simulink model "testrig_AirOilPiston"  (R2026b)
settings: Solver=daessc  StopTime=25  MaxStep=1e-3  AbsTol=1e-3
PreLoadFcn:
  | Spring = VDatabase.Spring.SUV_Landy_TA2PR_AirOilPiston_A1;
  | mass_sprung = 436.5;
  | load testrig_AirOilPiston_roughroad
PostLoadFcn:
  | warning off Simulink:blocks:TDelayBufferTooSmall
undefined symbols (not defined in the file or in its folder): Triangle
libraries: fl_lib x10, nesl_utility x5, simulink x4, Spring_AirOilPiston x1, testrig_AirOilPiston_lib x1
settings Model: Creator=Glenn  LastModifiedBy=smiller
settings SolverCC: AutoScaleAbsTol=off  MaxConsecutiveMinStep=5
settings DataIOCC: ReturnWorkspaceOutputs=off  SignalLoggingName=logsout_testrig_AirOilPiston
settings SimscapeCC: SimscapeLogLimitData=off  SimscapeLogName=simlog_testrig_AirOilPiston  SimscapeLogType=all  SimscapeUseEnergyAccounting=off

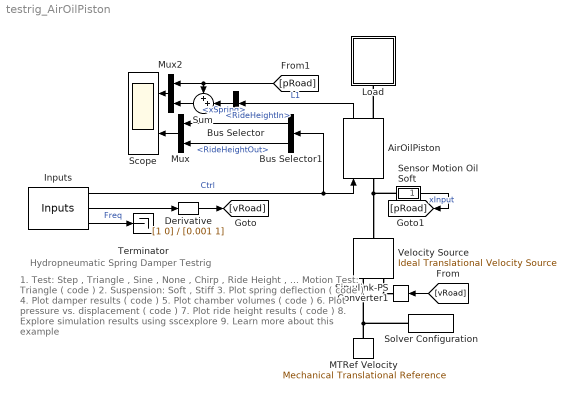
== system testrig_AirOilPiston ==
  note: 1. Test: Step , Triangle , Sine , None , Chirp , Ride Height , ... Motion Test: Triangle ( code )
      | 2. Suspension: Soft , Stiff
      | 3. Plot spring deflection ( code )
      | 4. Plot damper results ( code )
      | 5. Plot chamber volumes ( code )
      | 6. Plot pressure vs. displacement ( code )
      | 7. Plot ride height results ( code )
      | 8. Explore simulation results using sscexplore
      | 9. Learn more about this example
  note: Hydropneumatic Spring Damper Testrig
  AirOilPiston : Spring_AirOilPiston/AirOilPiston  spr_hp_top=Spring.sTop.Value*0  spr_hp_bot=Spring.sBottom.Value*0  t_ambient=Spring.Spring.TAmbient.Value  gspr_gas_properties=Spring.Spring.GasProperties  strut_oil_properties=Spring.Strut.OilProperties  gas_chamber_soft_area=Spring.Spring.GasSoft.A.Value  gas_chamber_stiff_area=Spring.Spring.GasStiff.A.Value  gas_chamber_soft_deadvol=Spring.Spring.GasSoft.volDead.Value  gas_chamber_stiff_deadvol=Spring.Spring.GasStiff.volDead.Value  gspr_mass_soft=Spring.Spring.GasSoft.mPiston.Value  gspr_mass_stiff=Spring.Spring.GasStiff.mPiston.Value  gspr_damping_soft=Spring.Spring.GasSoft.b.Value  gspr_damping_stiff=Spring.Spring.GasStiff.b.Value  gas_chamber_soft_x0=Spring.Spring.GasSoft.xInit.Value  gas_chamber_stiff_x0=Spring.Spring.GasStiff.xInit.Value  gas_chamber_soft_p0=Spring.Spring.GasSoft.pInit.Value  gas_chamber_stiff_p0=Spring.Spring.GasStiff.pInit.Value  gspr_cwall_soft=Spring.Spring.GasSoft.CWall.Value  gspr_cwall_stiff=Spring.Spring.GasStiff.CWall.Value  oil_chamber_soft_area=Spring.Spring.OilSoft.A.Value  oil_chamber_stiff_area=Spring.Spring.OilStiff.A.Value  oil_chamber_soft_deadvol=Spring.Spring.OilSoft.volDead.Value  oil_chamber_stiff_deadvol=Spring.Spring.OilStiff.volDead.Value  oil_chamber_soft_x0=Spring.Spring.OilSoft.xInit.Value  oil_chamber_stiff_x0=Spring.Spring.OilStiff.xInit.Value  oil_chamber_soft_p0=Spring.Spring.OilSoft.pInit.Value  oil_chamber_stiff_p0=Spring.Spring.OilStiff.pInit.Value  gsprv_smax_soft=Spring.Spring.ValveSoft.xMaxOpen.Value  gsprv_smax_stiff=Spring.Spring.ValveStiff.xMaxOpen.Value  gsprv_delsmax_soft=Spring.Spring.ValveSoft.xCloseToOpen.Value  gsprv_delsmax_stiff=Spring.Spring.ValveStiff.xCloseToOpen.Value  gsprv_arealeak_soft=Spring.Spring.ValveSoft.areaLeak.Value  gsprv_arealeak_stiff=Spring.Spring.ValveStiff.areaLeak.Value  gsprv_areamax_soft=Spring.Spring.ValveSoft.aMax.Value  gsprv_areamax_stiff=Spring.Spring.ValveStiff.aMax.Value  gsprv_cd_soft=Spring.Spring.ValveSoft.Cd.Value  gsprv_cd_stiff=Spring.Spring.ValveStiff.Cd.Value  gsprv_smooth_soft=Spring.Spring.ValveSoft.smoothFactor.Value  gsprv_smooth_stiff=Spring.Spring.ValveStiff.smoothFactor.Value  gsprva_stroke_soft=Spring.Spring.ValveActuatorSoft.xStroke.Value  gsprva_stroke_stiff=Spring.Spring.ValveActuatorStiff.xStroke.Value  gsprva_ton_soft=Spring.Spring.ValveActuatorSoft.tOn.Value  gsprva_ton_stiff=Spring.Spring.ValveActuatorStiff.tOn.Value  gsprva_toff_soft=Spring.Spring.ValveActuatorSoft.tOff.Value  gsprva_toff_stiff=Spring.Spring.ValveActuatorStiff.tOff.Value  strut_deadvol=Spring.Strut.volDead.Value  strut_area=Spring.Strut.A.Value  strut_x0=Spring.Strut.xInit.Value  strut_frc_colfrc=Spring.Strut.Friction.fCoulomb.Value  strut_frc_brkfrc=Spring.Strut.Friction.fBreakaway.Value  strut_frc_brkvel=Spring.Strut.Friction.vBreakaway.Value  strut_frc_visccoeff=Spring.Strut.Friction.mu.Value  strut_p0=Spring.Strut.pInit.Value  bs_lim_upper=Spring.Endstop.xMax.Value  bs_lim_lower=Spring.Endstop.xMin.Value  bs_k_upper=Spring.Endstop.KxMax.Value  bs_k_lower=Spring.Endstop.KxMin.Value  bs_b_upper=Spring.Endstop.dxMax.Value  bs_b_lower=Spring.Endstop.dxMin.Value  bs_region=Spring.Endstop.xTransition.Value  p_diff_TLU_constant=Spring.Damper.Orifice.pDiff.Value  vol_flow_TLU_constant=Spring.Damper.Orifice.q.Value  dpr_restrarea_comp=Spring.Damper.RestrictionComp.A.Value  dpr_restrarea_reb=Spring.Damper.RestrictionReb.A.Value  dpr_cd_comp=Spring.Damper.RestrictionComp.Cd.Value  dpr_cd_reb=Spring.Damper.RestrictionReb.Cd.Value  dpr_prv_psetdiff_comp=Spring.Damper.PRVComp.pDiff.Value  dpr_prv_psetdiff_reb=Spring.Damper.PRVReb.pDiff.Value  dpr_prv_prange_comp=Spring.Damper.PRVComp.pRange.Value  dpr_prv_prange_reb=Spring.Damper.PRVReb.pRange.Value  dpr_prv_areamax_comp=Spring.Damper.PRVComp.A.Value  dpr_prv_areamax_reb=Spring.Damper.PRVReb.A.Value  dpr_prv_cd_comp=Spring.Damper.PRVComp.Cd.Value  dpr_prv_cd_reb=Spring.Damper.PRVReb.Cd.Value  dpr_cvdvalve_cmpos=Spring.CVDValve.Orifice.x.Value  dpr_cvdvalve_orifice_area=Spring.CVDValve.Orifice.A.Value  dpr_cvdvalve_orifice_pdiff=Spring.CVDValve.Orifice.pDiff.Value  dpr_cvdvalve_pcv_areamax=Spring.CVDValve.PCValve.AMax.Value  dpr_cvdvalve_pcv_prange=Spring.CVDValve.PCValve.pRange.Value  dpr_cvdvalve_arealeak=Spring.CVDValve.PCValve.ALeak.Value  dpr_cvdvalve_cd=Spring.CVDValve.PCValve.Cd.Value  dpr_cvdvalve_act_ts=Spring.CVDValve.tFilt.Value  rh_srcpressure=Spring.RideHeight.pSource.Value  rh_fcv_cmpos_inlet=Spring.RideHeight.OrificeInlet.x.Value  rh_fcv_cmpos_outlet=Spring.RideHeight.OrificeOutlet.x.Value  rh_fcv_orificearea_inlet=Spring.RideHeight.OrificeInlet.A.Value  rh_fcv_orificearea_outlet=Spring.RideHeight.OrificeOutlet.A.Value  rh_fcv_orificepdiff_inlet=Spring.RideHeight.OrificeInlet.pDiff.Value  rh_fcv_orificepdiff_outlet=Spring.RideHeight.OrificeOutlet.pDiff.Value  rh_fcv_pcprange_inlet=Spring.RideHeight.PCValveInlet.pRange.Value  rh_fcv_pcprange_outlet=Spring.RideHeight.PCValveOutlet.pRange.Value  rh_fcv_pcamax_inlet=Spring.RideHeight.PCValveInlet.AMax.Value  rh_fcv_pcamax_outlet=Spring.RideHeight.PCValveOutlet.AMax.Value  rh_fcv_arealeak_inlet=Spring.RideHeight.PCValveInlet.ALeak.Value  rh_fcv_arealeak_outlet=Spring.RideHeight.PCValveOutlet.ALeak.Value  rh_fcv_cd_inlet=Spring.RideHeight.PCValveInlet.Cd.Value  rh_fcv_cd_outlet=Spring.RideHeight.PCValveOutlet.Cd.Value  rh_fcv_smooth_inlet=Spring.RideHeight.PCValveInlet.smoothFactor.Value  rh_fcv_smooth_outlet=Spring.RideHeight.PCValveOutlet.smoothFactor.Value  rh_fcv_tfilt_inlet=Spring.RideHeight.PCValveInlet.tFilt.Value  rh_fcv_tfilt_outlet=Spring.RideHeight.PCValveOutlet.tFilt.Value
  Bus Selector : BusSelector  OutputSignals=xSpring
  Bus Selector1 : BusSelector  OutputSignals=RideHeightIn,RideHeightOut
  Derivative : TransferFcn  Numerator=[1 0]  Denominator=[0.001 1]
  Inputs : testrig_AirOilPiston_lib/Inputs  popup_suspension_stiffness=Soft  popup_rh_test_seq=None  cvd_value=1  popup_roadpz_test_type=Step  pAmp=0.05  tPer=4  nCyc=50  nCycSet=1  chirpFreqFinish=10  chirpFreqStart=0.5  chirpTimeFinish=25  chirpTimeStart=5  spdkmh=10  roughTimeStart=5
      settings: AttributesFormatString=|
      | Road Height: %<popup_roadpz_test_type>
      | Suspension: %<popup_suspension_stiffness>
      | Ride Height: %<popup_rh_test_seq>
  Load : Subsystem  Variant=on  VariantControlMode=label  VariantControl=Mass  LabelModeActiveChoice=Mass  mask{popup_load_type=Mass}
      mask prompts: popup_load_type "Load Type"
      mask init:
      | bh = gcb;
      | set_param(gcb,'LabelModeActiveChoice',get_param(bh,'popup_load_type'));
      settings: AttributesFormatString=%<popup_load_type>
      mask TypeOptions popup_load_type: Mass | Motion
      mask Display: disp(' ')
  MTRef Velocity : fl_lib/Mechanical/Translational Elements/Mechanical Translational Reference
  Mux : Mux  Inputs=2
  Mux2 : Mux  Inputs=2
  Scope : Scope  NumInputPorts=2
      settings: ActiveDisplayYMinimum=-0.07527  ActiveDisplayYMaximum=0.08974
  Sensor Motion Oil Soft : Subsystem
  Simulink-PS Converter1 : nesl_utility/Simulink-PS Converter  PhysicalDomain=network_engine_domain  SubClassName=ps_input  LeftPortType=input  RightPortType=output  PseudoPeriodic=off  Frequencies=[]  NoiseDistribution=none  NoiseParameters=[]  Unit=m/s  AffineConversion=off  FilteringAndDerivatives=provide  SimscapeFilterOrder=1  InputFilterTimeConstant=0.001  UdotUserProvided=0
  Solver Configuration : nesl_utility/Solver Configuration  PhysicalDomain=network_engine_domain  SubClassName=solver  LeftPortType=input  RightPortType=generic  Tones=[]  Harmonics=[]  SimulateNoise=off  Profile=off  UseLocalSampling=off  EnableSwitchedLinearOptims=on  FrequencyDomain=off  UseCCode=off  RelTol=0.001  AbsTol=0.001  MinStep=1e-09  ToWorkspace=off  RevertToSquareIcSolve=off  NumHomotopyIterations=100  PhasorMode=off  PhasorModeNumHarmonics=1  ConsistencySolver=NEWTON_FTOL  CanonicalOrdering=UNORDERED  OptimizeIntermediates=UNOPTIMIZED  MulticoreSolverChoice=BACKWARD_EULER  IndexReductionMethod=DerivativeReplacement  DoDC=off  ResidualTolerance=1e-09  ConsistencyTolSource=GLOBAL  ConsistencyAbsTol=0.001  ConsistencyRelTol=0.001  ConsistencyTolFactor=0.001  UseLocalSolver=off  LocalSolverChoice=NE_BACKWARD_EULER_ADVANCER  ResolveIndetEquations=on  FunctionEvalNumThread=1  LocalSolverSampleTime=0.001  DoFixedCost=off  MaxNonlinIter=3  MaxModeIter=2  ComputeImpulses=off  ImpulseIterations=2  LinearAlgebra=auto  LinearAlgebraNumThread=0  EquationFormulation=NE_TIME_EF  DelaysMemoryBudget=1024  AutomaticFiltering=on  FilteringTimeConstant=0.001  PartitionStorageMethod=AS_NEEDED  PartitionMemoryBudget=1024  PartitionMethod=BALANCED  MultibodyUseLocalSolver=off  MultibodyLocalSolverChoice=ODE1  MultibodyLocalSolverSampleTime=0.001
  Sum : Sum  Inputs=++|
  Terminator : Terminator
  Velocity Source : fl_lib/Mechanical/Mechanical Sources/Ideal Translational Velocity Source
  wires:
  AirOilPiston/1 -> Bus Selector/1  "L1"
  Bus Selector/1 -> Sum/2  "<xSpring>"
  Mux/1 -> Scope/2
  Bus Selector1/1 -> Mux/1  "<RideHeightIn>"
  Bus Selector1/2 -> Mux/2  "<RideHeightOut>"
  Inputs/2 -> Derivative/1
  [vRoad] -> Simulink-PS Converter1/1
  Inputs/1 -> Bus Selector1/1, AirOilPiston/1  "Ctrl"
  Mux2/1 -> Scope/1
  Sensor Motion Oil Soft/1(P) -> [pRoad]  "xInput"
  Derivative/1 -> [vRoad]
  [pRoad] -> Sum/1, Mux2/1
  Sum/1 -> Mux2/2
  Inputs/3 -> Terminator/1  "Freq"
  connections:
  Sensor Motion Oil Soft/LConn1 -- AirOilPiston/LConn1 -- Velocity Source/LConn1
  MTRef Velocity/LConn1 -- Solver Configuration/RConn1 -- Velocity Source/RConn2
  Velocity Source/RConn1 -- Simulink-PS Converter1/RConn1
  AirOilPiston/RConn1 -- Load/LConn1

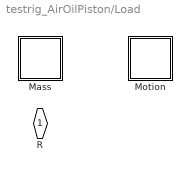
== system testrig_AirOilPiston/Load ==
  Mass : Subsystem  VariantControl=Mass
  Motion : Subsystem  VariantControl=Motion  mask{popup_signalType=Triangle, pAmp=0.05, tPer=3, nCyc=50, nCycSet=1, chirpFreqFinish=10, chirpFreqStart=0.5, chirpTimeFinish=20, chirpTimeStart=5}
      mask prompts: popup_signalType "Signal Type"; pAmp "Amplitude"; tPer "Period"; nCyc "Number of Cycles per Set"; nCycSet "Number of Cycles to Settle"; chirpFreqFinish "Chirp Freq Finish (Hz)"; chirpFreqStart "Chirp Freq Start (Hz)"; chirpTimeFinish "Chirp Time Finish (sec)"; chirpTimeStart "Chirp Start Delay (sec)"
      mask TypeOptions popup_signalType: Spring Extension Velocity/popup_signalType
      mask Callback popup_signalType:
      | bh = gcb;
      | maskObj = Simulink.Mask.get(bh); % Get the mask object of the current block
      | 
      | % Handles for parameter visibility
      | chFrSt_h  = maskObj.getParameter('chirpFreqStart'); % Get the parameter to hide
      | chFrFi_h  = maskObj.getParameter('chirpFreqFinish'); % Get the parameter to hide
      | chTiSt_h  = maskObj.getParameter('chirpTimeStart'); % Get the parameter to hide
      | chTiFi_h  = maskObj.getParameter('chirpTimeFinish'); % Get the parameter to hide
      | 
      | tPer_h    = maskObj.getParameter('tPer');    % Get the parameter to hide
      | nCycSet_h = maskObj.getParameter('nCycSet'); % Get the parameter to hide
      | nCyc_h    = maskObj.getParameter('nCyc'); % Get the parameter to hide
      | 
      | % Check the value of ControlParam
      | controlParamValue = get_param(bh, 'popup_signalType');
      | 
      | chFrSt_h.Visible   = 'off';
      | chFrFi_h.Visible   = 'off';
      | chTiFi_h.Visible   = 'off';
      | chTiSt_h.Visible   = 'off';
      | tPer_h.Visible     = 'on';
      | nCycSet_h.Visible  = 'on';
      | nCyc_h.Visible     = 'on';
      | 
      | if(strcmp(controlParamValue, 'Chirp'))
      |     chFrSt_h.Visible  = 'on';
      |     chFrFi_h.Visible  = 'on';
      |     chTiSt_h.Visible  = 'on';
      |     chTiFi_h.Visible  = 'on';
      | 
      |     tPer_h.Visible    = 'off';
      |     nCycSet_h.Visible = 'off';
      |     nCyc_h.Visible    = 'off';
      | end
      mask TypeOptions pAmp: Spring Extension Velocity/vAmp
      mask TypeOptions tPer: Spring Extension Velocity/tPer
      mask TypeOptions nCyc: Spring Extension Velocity/nCyc
      mask TypeOptions nCycSet: Spring Extension Velocity/nCycSet
      mask TypeOptions chirpFreqFinish: Spring Extension Velocity/chirpFreqFinish
      mask TypeOptions chirpFreqStart: Spring Extension Velocity/chirpFreqStart
      mask TypeOptions chirpTimeFinish: Spring Extension Velocity/chirpTimeFinish
      mask TypeOptions chirpTimeStart: Spring Extension Velocity/chirpTimeStart
  R : PMIOPort  Side=Left

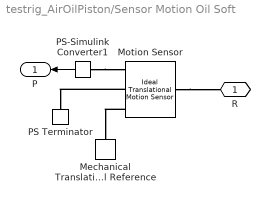
== system testrig_AirOilPiston/Sensor Motion Oil Soft ==
  Mechanical Translational Reference : fl_lib/Mechanical/Translational Elements/Mechanical Translational Reference
  Motion Sensor : fl_lib/Mechanical/Mechanical Sensors/Ideal Translational Motion Sensor  reference=foundation.enum.MeasurementReference.difference  acceleration_port=false  velocity_port=true  position_port=true  offset=0 m
  PS Terminator : fl_lib/Physical Signals/Sinks/PS Terminator
  PS-Simulink Converter1 : nesl_utility/PS-Simulink Converter  PhysicalDomain=network_engine_domain  SubClassName=ps_output  LeftPortType=input  RightPortType=output  PseudoPeriodic=off  Frequencies=[]  VectorFormat=inherit  Unit=m  AffineConversion=off
  R : PMIOPort  Side=Left
  P : Outport
  wires:
  PS-Simulink Converter1/1 -> P/1
  connections:
  PS-Simulink Converter1/LConn1 -- Motion Sensor/RConn3
  Motion Sensor/LConn1 -- R/RConn1
  Motion Sensor/RConn1 -- Mechanical Translational Reference/LConn1
  Motion Sensor/RConn2 -- PS Terminator/LConn1

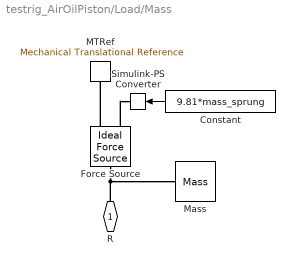
== system testrig_AirOilPiston/Load/Mass ==
  Constant : Constant  Value=9.81*mass_sprung
  Force Source : fl_lib/Mechanical/Mechanical Sources/Ideal Force Source
  MTRef : fl_lib/Mechanical/Translational Elements/Mechanical Translational Reference
  Mass : fl_lib/Mechanical/Translational Elements/Mass  mass=mass_sprung kg  num_ports=foundation.enum.numPorts2.one  v_specify=off  v_priority=High  v=0 m/s  v_nominal_specify=off  v_nominal_value=1  v_nominal_unit=m/s  f_specify=off  f_priority=None  f=0 N  f_nominal_specify=off  f_nominal_value=1  f_nominal_unit=N
  Simulink-PS Converter : nesl_utility/Simulink-PS Converter  PhysicalDomain=network_engine_domain  SubClassName=ps_input  LeftPortType=input  RightPortType=output  PseudoPeriodic=off  Frequencies=[]  NoiseDistribution=none  NoiseParameters=[]  Unit=1  AffineConversion=off  FilteringAndDerivatives=provide  SimscapeFilterOrder=1  InputFilterTimeConstant=0.001  UdotUserProvided=0
  R : PMIOPort  Side=Left
  wires:
  Constant/1 -> Simulink-PS Converter/1
  connections:
  Force Source/RConn1 -- Simulink-PS Converter/RConn1
  Force Source/RConn2 -- MTRef/LConn1
  R/RConn1 -- Force Source/LConn1 -- Mass/LConn1

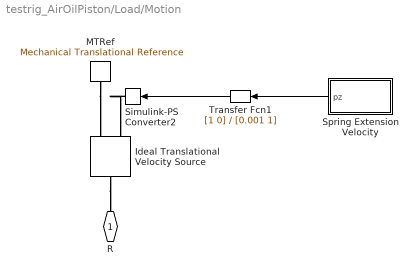
== system testrig_AirOilPiston/Load/Motion ==
  Ideal Translational Velocity Source : fl_lib/Mechanical/Mechanical Sources/Ideal Translational Velocity Source
  MTRef : fl_lib/Mechanical/Translational Elements/Mechanical Translational Reference
  Simulink-PS Converter2 : nesl_utility/Simulink-PS Converter  PhysicalDomain=network_engine_domain  SubClassName=ps_input  LeftPortType=input  RightPortType=output  PseudoPeriodic=off  Frequencies=[]  NoiseDistribution=none  NoiseParameters=[]  Unit=1  AffineConversion=off  FilteringAndDerivatives=filter  SimscapeFilterOrder=1  InputFilterTimeConstant=0.01  UdotUserProvided=0
  Spring Extension Velocity : Subsystem  mask{popup_signalType=Triangle, tPer=tPer, chirpFreqStart=chirpFreqStart, chirpFreqFinish=chirpFreqFinish, chirpTimeStart=chirpTimeStart, chirpTimeFinish=chirpTimeFinish, vAmp=pAmp, nCyc=nCyc, nCycSet=nCycSet}
      mask prompts: popup_signalType "Signal Type"; tPer "Period"; chirpFreqStart "Chirp Freq Start (Hz)"; chirpFreqFinish "Chirp Freq Finish (Hz)"; chirpTimeStart "Chirp Start Delay (sec)"; chirpTimeFinish "Chirp Time Finish (sec)"; vAmp "Amplitude"; nCyc "Number of Cycles per Set"; nCycSet "Number of Cycles to Settle"
      mask init:
      | bh = gcb;
      | 
      | sigType = get_param(bh,'popup_signalType');
      | set_param([bh '/Velocity Signal'],'LabelModeActiveChoice',sigType)
      | 
      | pVec_time  = [0 tPer/4 tPer/2 3*tPer/4 tPer];
      | pVec_val_Cyc = [0 1 0 -1 0];
      | 
      | sVec_time  = [0 0.05 0.5 0.55 0.95 1]*tPer;
      | sVec_val_Cyc = [0 1 1 0 0 0];
      | 
      | iVec_time    = [0 0.25 0.27 0.29 0.31 0.75  0.77  0.79 0.81 1]*tPer;
      | iVec_val_Cyc = [0 0    1    1    0    0    -1    -1    0    0];
      | 
      | %qVec_time     = [0 tPer/4 tPer/2 3*tPer/4 tPer]*tPer;
      | %qVec_val_Cyc  = [0 1 0 -1 0];
      | 
      | 
      | %aVec_time  = [0 [0 tPer/2 nCyc*tPer+[-1 0]*tPer/2]+nCycSet*tPer];
      | aVec_time  = [0 [0 1e-3 nCyc*tPer+[-1 0]*1e-3]+nCycSet*tPer];
      | 
      | if(strcmp(sigType,'Chirp'))
      |     aVec_value = [1 1 1 1 1];
      | else
      |     aVec_value = [0 0 1 1 0];
      | end
      settings: AttributesFormatString=%<popup_signalType>
      mask TypeOptions popup_signalType: Sine | Triangle | Pulse | None | Chirp
      mask Callback popup_signalType:
      | bh = gcb;
      | maskObj = Simulink.Mask.get(bh); % Get the mask object of the current block
      | 
      | % Handles for parameter visibility
      | chFrSt_h  = maskObj.getParameter('chirpFreqStart'); % Get the parameter to hide
      | chFrFi_h  = maskObj.getParameter('chirpFreqFinish'); % Get the parameter to hide
      | chTiSt_h  = maskObj.getParameter('chirpTimeStart'); % Get the parameter to hide
      | chTiFi_h  = maskObj.getParameter('chirpTimeFinish'); % Get the parameter to hide
      | 
      | tPer_h    = maskObj.getParameter('tPer');    % Get the parameter to hide
      | nCycSet_h = maskObj.getParameter('nCycSet'); % Get the parameter to hide
      | nCyc_h    = maskObj.getParameter('nCyc'); % Get the parameter to hide
      | 
      | % Check the value of ControlParam
      | controlParamValue = get_param(bh, 'popup_signalType');
      | 
      | chFrSt_h.Visible   = 'off';
      | chFrFi_h.Visible   = 'off';
      | chTiFi_h.Visible   = 'off';
      | chTiSt_h.Visible   = 'off';
      | tPer_h.Visible     = 'on';
      | nCycSet_h.Visible  = 'on';
      | nCyc_h.Visible     = 'on';
      | 
      | if(strcmp(controlParamValue, 'Chirp'))
      |     chFrSt_h.Visible  = 'on';
      |     chFrFi_h.Visible  = 'on';
      |     chTiSt_h.Visible  = 'on';
      |     chTiFi_h.Visible  = 'on';
      | 
      |     tPer_h.Visible    = 'off';
      |     nCycSet_h.Visible = 'off';
      |     nCyc_h.Visible    = 'off';
      | end
  Transfer Fcn1 : TransferFcn  Numerator=[1 0]  Denominator=[0.001 1]
  R : PMIOPort  Side=Left
  wires:
  Spring Extension Velocity/1(pz) -> Transfer Fcn1/1
  Transfer Fcn1/1 -> Simulink-PS Converter2/1
  connections:
  MTRef/LConn1 -- Ideal Translational Velocity Source/RConn2
  Simulink-PS Converter2/RConn1 -- Ideal Translational Velocity Source/RConn1
  Ideal Translational Velocity Source/LConn1 -- R/RConn1

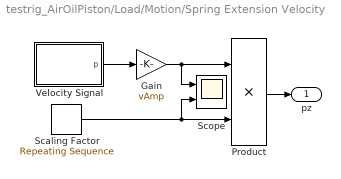
== system testrig_AirOilPiston/Load/Motion/Spring Extension Velocity ==
  Gain : Gain  Gain=vAmp
  Product : Product
  Scaling Factor : simulink/Sources/Repeating Sequence  rep_seq_t=aVec_time  rep_seq_y=aVec_value
  Scope : Scope  NumInputPorts=2
      settings: ActiveDisplayYMinimum=-0.015  ActiveDisplayYMaximum=0.135
  Velocity Signal : Subsystem  Variant=on  VariantControlMode=label  VariantControl=Sine  LabelModeActiveChoice=Triangle
  pz : Outport
  wires:
  Scaling Factor/1 -> Scope/2, Product/2
  Product/1 -> pz/1
  Velocity Signal/1(p) -> Gain/1
  Gain/1 -> Product/1, Scope/1

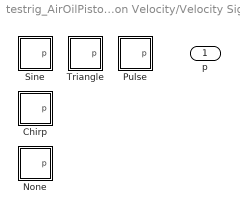
== system testrig_AirOilPiston/Load/Motion/Spring Extension Velocity/Velocity Signal ==
  Chirp : Subsystem  VariantControl=Chirp
  None : Subsystem  VariantControl=None
  Pulse : Subsystem  VariantControl=Pulse
  Sine : Subsystem  VariantControl=Sine
  Triangle : Subsystem  VariantControl=Triangle
  p : Outport

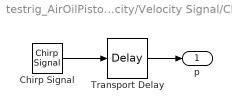
== system testrig_AirOilPiston/Load/Motion/Spring Extension Velocity/Velocity Signal/Chirp ==
  Chirp Signal : simulink/Sources/Chirp Signal  f1=chirpFreqStart  T=chirpTimeFinish  f2=chirpFreqFinish
  Transport Delay : TransportDelay  DelayTime=chirpTimeStart  BufferSize=5120
  p : Outport
  wires:
  Chirp Signal/1 -> Transport Delay/1
  Transport Delay/1 -> p/1

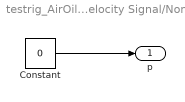
== system testrig_AirOilPiston/Load/Motion/Spring Extension Velocity/Velocity Signal/None ==
  Constant : Constant  Value=0
  p : Outport
  wires:
  Constant/1 -> p/1

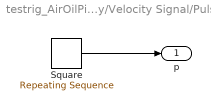
== system testrig_AirOilPiston/Load/Motion/Spring Extension Velocity/Velocity Signal/Pulse ==
  Square : simulink/Sources/Repeating Sequence  rep_seq_t=sVec_time  rep_seq_y=sVec_val_Cyc
  p : Outport
  wires:
  Square/1 -> p/1

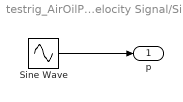
== system testrig_AirOilPiston/Load/Motion/Spring Extension Velocity/Velocity Signal/Sine ==
  Sine Wave : Sin  Bias=1  Frequency=2*pi/tPer  Phase=-pi/2  SampleTime=0
  p : Outport
  wires:
  Sine Wave/1 -> p/1

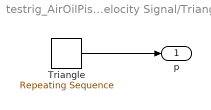
== system testrig_AirOilPiston/Load/Motion/Spring Extension Velocity/Velocity Signal/Triangle ==
  Triangle : simulink/Sources/Repeating Sequence  rep_seq_t=pVec_time  rep_seq_y=pVec_val_Cyc
  p : Outport
  wires:
  Triangle/1 -> p/1
